simulink subsystem "TestSubsystem"  (R2026a)
settings: Solver=VariableStepAuto
settings Model: Creator=wyatt  LastModifiedBy=wyatt

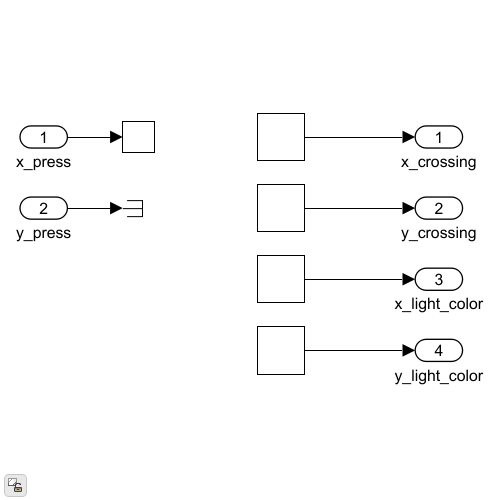
[thumbnail: Simulink's stored preview of the top-level diagram]
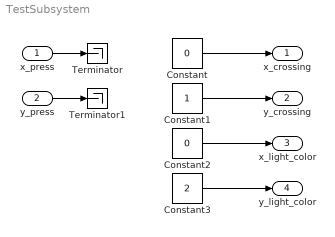
== system TestSubsystem ==
  x_press : Inport  OutDataTypeStr=boolean
  y_press : Inport  Port=2  OutDataTypeStr=boolean
  Constant : Constant  Value=0  OutDataTypeStr=boolean
  Constant1 : Constant  OutDataTypeStr=boolean
  Constant2 : Constant  Value=0  OutDataTypeStr=int8
  Constant3 : Constant  Value=2  OutDataTypeStr=int8
  Terminator : Terminator
  Terminator1 : Terminator
  x_crossing : Outport  OutDataTypeStr=boolean
  y_crossing : Outport  Port=2  OutDataTypeStr=boolean
  x_light_color : Outport  Port=3  OutDataTypeStr=int8
  y_light_color : Outport  Port=4  OutDataTypeStr=int8
  wires:
  x_press/1 -> Terminator/1
  y_press/1 -> Terminator1/1
  Constant1/1 -> y_crossing/1
  Constant/1 -> x_crossing/1
  Constant3/1 -> y_light_color/1
  Constant2/1 -> x_light_color/1
